simulink model "IEEE9BusSystem_eval"  (R2024a)
settings: Solver=FixedStepAuto  StartTime=0  StopTime=100  FixedStep=Ts  RelTol=1e-3  AbsTol=1e-3  EnableMultiTasking=on
PreLoadFcn:
  | Ts = 1/60;
libraries: ee_lib x63, nesl_utility x48, fl_lib x22, eeGeneralControl x6, spsFrequencyPhasorLib x3, eeSmAC1C x3, eeSmPSS1A x3, spspowerguiLib x1
(part 1 of 2)
Description:
  | IEEE 9-Bus System
settings Model: Creator=The MathWorks, Inc.  LastModifiedBy=yushixuan
settings SolverCC: AutoScaleAbsTol=off  AlgebraicLoopSolver=TrustRegion
settings DataIOCC: MaxDataPoints=110000  SaveOutput=off  DSMLogging=off  SaveTime=off  ReturnWorkspaceOutputs=off  SignalLoggingName=logsout_IEEE9BusLoadflow
settings OptimizationCC: ReuseModelBlockBuffer=off  LifeSpan=inf
settings DebuggingCC: UnderspecifiedInitializationDetection=Classic  MergeDetectMultiDrivingBlocksExec=none  MaxConsecutiveZCsMsg=warning  UnconnectedInputMsg=warning  UnconnectedOutputMsg=warning  UnconnectedLineMsg=warning  SFUnexpectedBacktrackingDiag=warning  SFNoUnconditionalDefaultTransitionDiag=warning  SFExecutionAtInitializationDiag=none  ArithmeticOperatorsInVariantConditions=warning
settings ModelReferenceCC: EnableRefExpFcnMdlSchedulingChecks=on
settings SFSimCC: SimUseLocalCustomCode=off
settings RTWCC: RTWUseLocalCustomCode=off  GPUComputeCapability=3.5
settings CodeAppCC: StateflowObjectComments=on
settings GRTTargetCC: TargetLangStandard=C89/C90 (ANSI)
settings ConfigComp: CovMetricSettings=dw  CovSaveCumulativeToWorkspaceVar=on  CovSaveSingleToWorkspaceVar=on  CovExternalEMLEnable=off
settings SimscapeCC: SimscapeNormalizeSystem=off  SimscapeLogType=all  SimscapeLogName=simlog_IEEE9BusSystem  SimscapeLogLimitData=off  SimscapeOperatingPoint=op

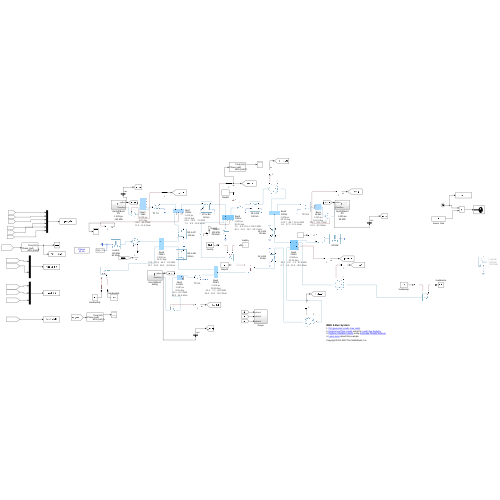
[thumbnail: Simulink's stored preview of the top-level diagram]
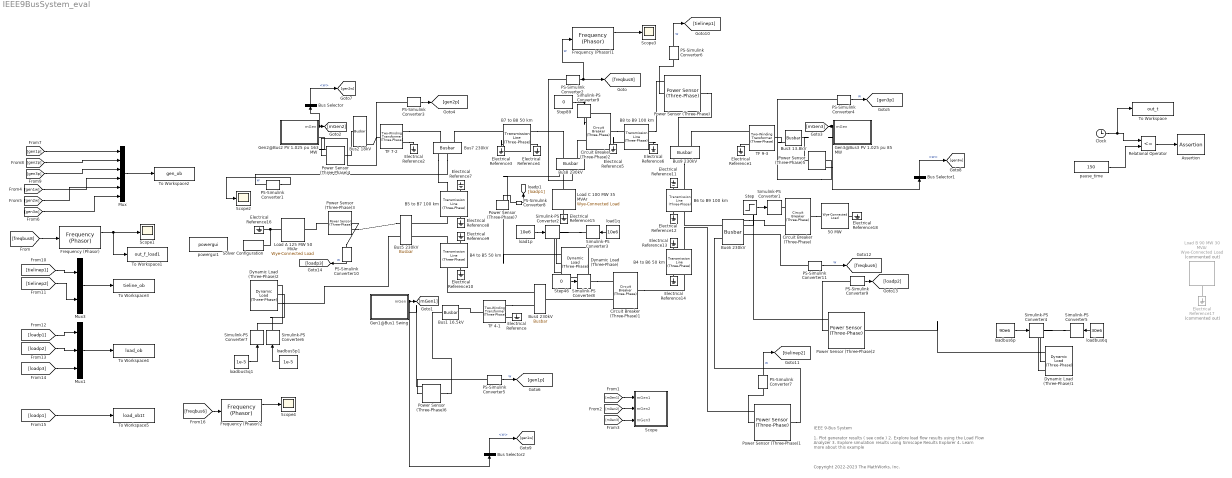
== system IEEE9BusSystem_eval ==
  note: Copyright 2022-2023 The MathWorks, Inc.
  note: 1. Plot generator results ( see code )
      | 2. Explore load flow results using the Load Flow Analyzer
      | 3. Explore simulation results using Simscape Results Explorer
      | 4. Learn more about this example
  note: IEEE 9-Bus System
  50 MW : ee_lib/Passive/RLC Assemblies/Wye-Connected Load  parameterization=2  component_structure=1  component_structure_PQ=1  R=1 Ohm  L=0.001 H  C=1e-6 F  VRated=230 kV  FRated=60 Hz  P=50 MW  Qpos=30e6 V*A  Qneg=-100 V*A  R_parasitic=1e-6 Ohm  G_parasitic=1e-6 1/Ohm  R_parasitic_PQ=1e-6 Ohm  G_parasitic_PQ=1e-6*0 1/Ohm  Vmag0=230e3 V  Vang0=0 rad  Freq0=60 Hz  IL_specify=on  IL_priority=High  IL=[ 0 0 0 ] A  IL_nominal_specify=off  IL_nominal_value=1  IL_nominal_unit=A  VC_specify=on  VC_priority=High  VC=[ 0 0 0 ] V  VC_nominal_specify=off  VC_nominal_value=1  VC_nominal_unit=V
  Assertion : Assertion  AssertionFailFcn=set_param(bdroot,'SimulationCommand','pause')  StopWhenAssertionFail=off
  B4 to B5 50 km : ee_lib/Passive/Lines/Transmission Line (Three-Phase)  length=50 km  freq=60 Hz  R=0.199333 Ohm/km  L=2.9658 mH/km  M=0.5803 mH/km  Cl=3.300e-3 uF/km  Cg=7.751e-3 uF/km  Rm=0.093533 Ohm/km  ModelTwoSections=ee.enum.enable.no  N=1  InterfacePosition=1 km  N1sec=1  N2sec=1  Access_ground=ee.enum.enable.no  R_parasitic=1e-6 Ohm  G_parasitic=1e-6 1/Ohm  EnableFault=false  fault_type_option=ee.enum.fault_type_option.ag  R_pn_fault=1e-3 Ohm  R_ng_fault=1e-3 Ohm  unfaulted_G_parasitic=1e-6 1/Ohm
      settings: InternalSimscapePortConfiguration="{\"Bottom\":[],\"Left\":[{\"id\":\"N1\",\"label\":\"~1\",\"type\":\"foundation.electrical.three_phase\"},{\"id\":\"g1\",\"label\":\"g1\",\"type\":\"foundation.electrical.electrical\"}],\"Right\":[{\"id\":\"N2\",\"label\":\"~2\",\"type\":\"foundation.electrical.three_phase\"},{\"id\":\"g2\",\"label\":\"g2\",\"type\":\"foundation.electrical.electrical\"}],\"Top\":[]}"
  B4 to B6 50 km : ee_lib/Passive/Lines/Transmission Line (Three-Phase)  length=50 km  freq=60 Hz  R=0.248707 Ohm/km  L=3.0967 mH/km  M=0.5148 mH/km  Cl=2.698e-3 uF/km  Cg=7.751e-3 uF/km  Rm=0.068847 Ohm/km  ModelTwoSections=ee.enum.enable.no  N=1  InterfacePosition=1 km  N1sec=1  N2sec=1  Access_ground=ee.enum.enable.no  R_parasitic=1e-6 Ohm  G_parasitic=1e-6 1/Ohm  EnableFault=false  fault_type_option=ee.enum.fault_type_option.ag  R_pn_fault=1e-3 Ohm  R_ng_fault=1e-3 Ohm  unfaulted_G_parasitic=1e-6 1/Ohm
      settings: InternalSimscapePortConfiguration="{\"Bottom\":[],\"Left\":[{\"id\":\"N1\",\"label\":\"~1\",\"type\":\"foundation.electrical.three_phase\"},{\"id\":\"g1\",\"label\":\"g1\",\"type\":\"foundation.electrical.electrical\"}],\"Right\":[{\"id\":\"N2\",\"label\":\"~2\",\"type\":\"foundation.electrical.three_phase\"},{\"id\":\"g2\",\"label\":\"g2\",\"type\":\"foundation.electrical.electrical\"}],\"Top\":[]}"
  B5 to B7 100 km : ee_lib/Passive/Lines/Transmission Line (Three-Phase)  length=100 km  freq=60 Hz  R=0.24165 Ohm/km  L=2.8816 mH/km  M=0.6224 mH/km  Cl=2.531e-3 uF/km  Cg=7.751e-3 uF/km  Rm=0.07237 Ohm/km  ModelTwoSections=ee.enum.enable.no  N=1  InterfacePosition=1 km  N1sec=1  N2sec=1  Access_ground=ee.enum.enable.no  R_parasitic=1e-6 Ohm  G_parasitic=1e-6 1/Ohm  EnableFault=false  fault_type_option=ee.enum.fault_type_option.ag  R_pn_fault=1e-3 Ohm  R_ng_fault=1e-3 Ohm  unfaulted_G_parasitic=1e-6 1/Ohm
      settings: InternalSimscapePortConfiguration="{\"Bottom\":[],\"Left\":[{\"id\":\"N1\",\"label\":\"~1\",\"type\":\"foundation.electrical.three_phase\"},{\"id\":\"g1\",\"label\":\"g1\",\"type\":\"foundation.electrical.electrical\"}],\"Right\":[{\"id\":\"N2\",\"label\":\"~2\",\"type\":\"foundation.electrical.three_phase\"},{\"id\":\"g2\",\"label\":\"g2\",\"type\":\"foundation.electrical.electrical\"}],\"Top\":[]}"
  B6 to B9 100 km : ee_lib/Passive/Lines/Transmission Line (Three-Phase)  length=100 km  freq=60 Hz  R=0.26634 Ohm/km  L=2.9658 mH/km  M=0.5803 mH/km  Cl=3.400e-3 uF/km  Cg=7.751e-3 uF/km  Rm=0.06003 Ohm/km  ModelTwoSections=ee.enum.enable.no  N=1  InterfacePosition=1 km  N1sec=1  N2sec=1  Access_ground=ee.enum.enable.no  R_parasitic=1e-6 Ohm  G_parasitic=1e-6 1/Ohm  EnableFault=false  fault_type_option=ee.enum.fault_type_option.ag  R_pn_fault=1e-3 Ohm  R_ng_fault=1e-3 Ohm  unfaulted_G_parasitic=1e-6 1/Ohm
      settings: InternalSimscapePortConfiguration="{\"Bottom\":[],\"Left\":[{\"id\":\"N1\",\"label\":\"~1\",\"type\":\"foundation.electrical.three_phase\"},{\"id\":\"g1\",\"label\":\"g1\",\"type\":\"foundation.electrical.electrical\"}],\"Right\":[{\"id\":\"N2\",\"label\":\"~2\",\"type\":\"foundation.electrical.three_phase\"},{\"id\":\"g2\",\"label\":\"g2\",\"type\":\"foundation.electrical.electrical\"}],\"Top\":[]}"
  B7 to B8 50 km : ee_lib/Passive/Lines/Transmission Line (Three-Phase)  length=50 km  freq=60 Hz  R=0.18875 Ohm/km  L=2.7226 mH/km  M=0.7019 mH/km  Cl=2.731e-3 uF/km  Cg=6.751e-3 uF/km  Rm=0.09882 Ohm/km  ModelTwoSections=ee.enum.enable.no  N=1  InterfacePosition=1 km  N1sec=1  N2sec=1  Access_ground=ee.enum.enable.no  R_parasitic=1e-6 Ohm  G_parasitic=1e-6 1/Ohm  EnableFault=false  fault_type_option=ee.enum.fault_type_option.ag  R_pn_fault=1e-3 Ohm  R_ng_fault=1e-3 Ohm  unfaulted_G_parasitic=1e-6 1/Ohm
      settings: InternalSimscapePortConfiguration="{\"Bottom\":[],\"Left\":[{\"id\":\"N1\",\"label\":\"~1\",\"type\":\"foundation.electrical.three_phase\"},{\"id\":\"g1\",\"label\":\"g1\",\"type\":\"foundation.electrical.electrical\"}],\"Right\":[{\"id\":\"N2\",\"label\":\"~2\",\"type\":\"foundation.electrical.three_phase\"},{\"id\":\"g2\",\"label\":\"g2\",\"type\":\"foundation.electrical.electrical\"}],\"Top\":[]}"
  B8 to B9 100 km : ee_lib/Passive/Lines/Transmission Line (Three-Phase)  length=100 km  freq=60 Hz  R=0.17077 Ohm/km  L=2.3184 mH/km  M=0.9040 mH/km  Cl=9.097e-4 uF/km  Cg=7.751e-3 uF/km  Rm=0.10782 Ohm/km  ModelTwoSections=ee.enum.enable.no  N=1  InterfacePosition=1 km  N1sec=1  N2sec=1  Access_ground=ee.enum.enable.no  R_parasitic=1e-6 Ohm  G_parasitic=1e-6 1/Ohm  EnableFault=false  fault_type_option=ee.enum.fault_type_option.ag  R_pn_fault=1e-3 Ohm  R_ng_fault=1e-3 Ohm  unfaulted_G_parasitic=1e-6 1/Ohm
      settings: InternalSimscapePortConfiguration="{\"Bottom\":[],\"Left\":[{\"id\":\"N1\",\"label\":\"~1\",\"type\":\"foundation.electrical.three_phase\"},{\"id\":\"g1\",\"label\":\"g1\",\"type\":\"foundation.electrical.electrical\"}],\"Right\":[{\"id\":\"N2\",\"label\":\"~2\",\"type\":\"foundation.electrical.three_phase\"},{\"id\":\"g2\",\"label\":\"g2\",\"type\":\"foundation.electrical.electrical\"}],\"Top\":[]}"
  Bus Selector : BusSelector  OutputSignals=w
  Bus Selector1 : BusSelector  OutputSignals=w
  Bus Selector2 : BusSelector  OutputSignals=w
  Bus1 16.5kV : ee_lib/Connectors & References/Busbar  Tag="1.040 pu\\n0.00 deg\\n42.4  -42.4 MW\\n38.5  -38.5 Mvar"  n_nodes=ee.enum.connectors.busbar_number_of_connections.two  VRated=16.5 kV  freq=60 Hz  show_ps=ee.enum.connectors.busbar_measurement.true
      settings: AttributesFormatString=%<Tag>  InternalSimscapePortConfiguration="{\"Bottom\":[],\"Left\":[{\"id\":\"N1\",\"label\":\"~1\",\"type\":\"foundation.electrical.three_phase\"}],\"Right\":[{\"id\":\"N2\",\"label\":\"~2\",\"type\":\"foundation.electrical.three_phase\"},{\"id\":\"Vt_ps\",\"label\":\"Vt\",\"type\":\"output\"},{\"id\":\"ph_ps\",\"label\":\"ph\",\"type\":\"output\"},{\"id\":\"P2_ps\",\"label\":\"P\",\"type\":\"output\"},{\"id\":\"Q2_ps\",\"label\":\"Q\",\"type\":\"output\"}],\"Top\":[]}"
  Bus2 18kV : ee_lib/Connectors & References/Busbar  Tag="1.025 pu\\n6.07 deg\\n83.2  -83.2 MW\\n11.5  -11.5 Mvar"  n_nodes=ee.enum.connectors.busbar_number_of_connections.two  VRated=18 kV  freq=60 Hz  show_ps=ee.enum.connectors.busbar_measurement.true
      settings: AttributesFormatString=%<Tag>  InternalSimscapePortConfiguration="{\"Bottom\":[],\"Left\":[{\"id\":\"N1\",\"label\":\"~1\",\"type\":\"foundation.electrical.three_phase\"}],\"Right\":[{\"id\":\"N2\",\"label\":\"~2\",\"type\":\"foundation.electrical.three_phase\"},{\"id\":\"Vt_ps\",\"label\":\"Vt\",\"type\":\"output\"},{\"id\":\"ph_ps\",\"label\":\"ph\",\"type\":\"output\"},{\"id\":\"P2_ps\",\"label\":\"P\",\"type\":\"output\"},{\"id\":\"Q2_ps\",\"label\":\"Q\",\"type\":\"output\"}],\"Top\":[]}"
  Bus3 13.8kV : ee_lib/Connectors & References/Busbar  Tag="1.025 pu\\n15.16 deg\\n201.7 -201.7 MW\\n10.9  -10.9 Mvar"  n_nodes=ee.enum.connectors.busbar_number_of_connections.two  VRated=13.8 kV  freq=60 Hz  show_ps=ee.enum.connectors.busbar_measurement.true
      settings: AttributesFormatString=%<Tag>  InternalSimscapePortConfiguration="{\"Bottom\":[],\"Left\":[{\"id\":\"N1\",\"label\":\"~1\",\"type\":\"foundation.electrical.three_phase\"}],\"Right\":[{\"id\":\"N2\",\"label\":\"~2\",\"type\":\"foundation.electrical.three_phase\"},{\"id\":\"Vt_ps\",\"label\":\"Vt\",\"type\":\"output\"},{\"id\":\"ph_ps\",\"label\":\"ph\",\"type\":\"output\"},{\"id\":\"P2_ps\",\"label\":\"P\",\"type\":\"output\"},{\"id\":\"Q2_ps\",\"label\":\"Q\",\"type\":\"output\"}],\"Top\":[]}"
  Bus4 230kV : ee_lib/Connectors & References/Busbar  Tag="1.019 pu\\n28.69 deg\\n42.2    7.2  -49.4 MW\\n36.5  -16.3  -20.2 Mvar"  n_nodes=ee.enum.connectors.busbar_number_of_connections.three  VRated=230 kV  freq=60 Hz  show_ps=ee.enum.connectors.busbar_measurement.false
      settings: AttributesFormatString=%<Tag>  InternalSimscapePortConfiguration="{\"Bottom\":[],\"Left\":[{\"id\":\"N1\",\"label\":\"~1\",\"type\":\"foundation.electrical.three_phase\"},{\"id\":\"N3\",\"label\":\"~3\",\"type\":\"foundation.electrical.three_phase\"}],\"Right\":[{\"id\":\"N2\",\"label\":\"~2\",\"type\":\"foundation.electrical.three_phase\"}],\"Top\":[]}"
  Bus5 230kV : ee_lib/Connectors & References/Busbar  Tag="0.990 pu\\n26.47 deg\\n73.5 -122.6   49.1   -0.0 MW\\n13.7  -49.0   35.3   -0.0 Mvar"  n_nodes=ee.enum.connectors.busbar_number_of_connections.four  VRated=230 kV  freq=60 Hz  show_ps=ee.enum.connectors.busbar_measurement.false
      settings: AttributesFormatString=%<Tag>  InternalSimscapePortConfiguration="{\"Bottom\":[],\"Left\":[{\"id\":\"N1\",\"label\":\"~1\",\"type\":\"foundation.electrical.three_phase\"},{\"id\":\"N3\",\"label\":\"~3\",\"type\":\"foundation.electrical.three_phase\"}],\"Right\":[{\"id\":\"N2\",\"label\":\"~2\",\"type\":\"foundation.electrical.three_phase\"},{\"id\":\"N4\",\"label\":\"~4\",\"type\":\"foundation.electrical.three_phase\"}],\"Top\":[]}"
  Bus6 230kV : ee_lib/Connectors & References/Busbar  Tag="0.998 pu\\n29.30 deg\\n95.1   -0.0   -7.3  -87.8 MW\\n3.7   -0.0   31.8  -35.5 Mvar"  n_nodes=ee.enum.connectors.busbar_number_of_connections.four  VRated=230 kV  freq=60 Hz  show_ps=ee.enum.connectors.busbar_measurement.true
      settings: AttributesFormatString=%<Tag>  InternalSimscapePortConfiguration="{\"Bottom\":[],\"Left\":[{\"id\":\"N1\",\"label\":\"~1\",\"type\":\"foundation.electrical.three_phase\"},{\"id\":\"N3\",\"label\":\"~3\",\"type\":\"foundation.electrical.three_phase\"}],\"Right\":[{\"id\":\"N2\",\"label\":\"~2\",\"type\":\"foundation.electrical.three_phase\"},{\"id\":\"N4\",\"label\":\"~4\",\"type\":\"foundation.electrical.three_phase\"},{\"id\":\"Vt_ps\",\"label\":\"Vt\",\"type\":\"output\"},{\"id\":\"ph_ps\",\"label\":\"ph\",\"type\":\"output\"},{\"id\":\"P4_ps\",\"label\":\"P\",\"type\":\"output\"},{\"id\":\"Q4_ps\",\"label\":\"Q\",\"type\":\"output\"}],\"Top\":[]}"
  Bus7 230kV : ee_lib/Connectors & References/Busbar  Tag="1.019 pu\\n33.23 deg\\n82.9  -75.3   -7.6 MW\\n7.2    8.3  -15.4 Mvar"  n_nodes=ee.enum.connectors.busbar_number_of_connections.three  VRated=230 kV  freq=60 Hz  show_ps=ee.enum.connectors.busbar_measurement.true
      settings: AttributesFormatString=%<Tag>  InternalSimscapePortConfiguration="{\"Bottom\":[],\"Left\":[{\"id\":\"N1\",\"label\":\"~1\",\"type\":\"foundation.electrical.three_phase\"},{\"id\":\"N3\",\"label\":\"~3\",\"type\":\"foundation.electrical.three_phase\"}],\"Right\":[{\"id\":\"N2\",\"label\":\"~2\",\"type\":\"foundation.electrical.three_phase\"},{\"id\":\"Vt_ps\",\"label\":\"Vt\",\"type\":\"output\"},{\"id\":\"ph_ps\",\"label\":\"ph\",\"type\":\"output\"},{\"id\":\"P3_ps\",\"label\":\"P\",\"type\":\"output\"},{\"id\":\"Q3_ps\",\"label\":\"Q\",\"type\":\"output\"}],\"Top\":[]}"
  Bus8 230kV : ee_lib/Connectors & References/Busbar  Tag="1.002 pu\\n33.03 deg\\n7.6   -8.6  101.4 -100.5 MW\\n30.2  -11.3   16.2  -35.1 Mvar"  n_nodes=ee.enum.connectors.busbar_number_of_connections.four  VRated=230 kV  freq=60 Hz  show_ps=ee.enum.connectors.busbar_measurement.true
      settings: AttributesFormatString=%<Tag>  InternalSimscapePortConfiguration="{\"Bottom\":[],\"Left\":[{\"id\":\"N1\",\"label\":\"~1\",\"type\":\"foundation.electrical.three_phase\"},{\"id\":\"N3\",\"label\":\"~3\",\"type\":\"foundation.electrical.three_phase\"}],\"Right\":[{\"id\":\"N2\",\"label\":\"~2\",\"type\":\"foundation.electrical.three_phase\"},{\"id\":\"N4\",\"label\":\"~4\",\"type\":\"foundation.electrical.three_phase\"},{\"id\":\"Vt_ps\",\"label\":\"Vt\",\"type\":\"output\"},{\"id\":\"ph_ps\",\"label\":\"ph\",\"type\":\"output\"},{\"id\":\"P4_ps\",\"label\":\"P\",\"type\":\"output\"},{\"id\":\"Q4_ps\",\"label\":\"Q\",\"type\":\"output\"}],\"Top\":[]}"
  Bus9 230kV : ee_lib/Connectors & References/Busbar  Tag="1.025 pu\\n38.70 deg\\n-102.7  -98.7  201.4 MW\\n-5.1   17.2  -12.1 Mvar"  n_nodes=ee.enum.connectors.busbar_number_of_connections.three  VRated=230 kV  freq=60 Hz  show_ps=ee.enum.connectors.busbar_measurement.false
      settings: AttributesFormatString=%<Tag>  InternalSimscapePortConfiguration="{\"Bottom\":[],\"Left\":[{\"id\":\"N1\",\"label\":\"~1\",\"type\":\"foundation.electrical.three_phase\"},{\"id\":\"N3\",\"label\":\"~3\",\"type\":\"foundation.electrical.three_phase\"}],\"Right\":[{\"id\":\"N2\",\"label\":\"~2\",\"type\":\"foundation.electrical.three_phase\"}],\"Top\":[]}"
  Circuit Breaker (Three-Phase) : ee_lib/Switches & Breakers/Circuit Breaker (Three-Phase)  R_closed=0.001 Ohm  G_open=1e-8 1/Ohm  threshold=0.5 V  breaker_behavior=ee.enum.switches.breakerBehavior.zeroCrossingDisable
      settings: InternalSimscapePortConfiguration="{\"Bottom\":[],\"Left\":[{\"id\":\"vT\",\"label\":\"vT\",\"type\":\"input\"},{\"id\":\"N1\",\"label\":\"~1\",\"type\":\"foundation.electrical.three_phase\"}],\"Right\":[{\"id\":\"N2\",\"label\":\"~2\",\"type\":\"foundation.electrical.three_phase\"}],\"Top\":[]}"
  Circuit Breaker (Three-Phase)1 : ee_lib/Switches & Breakers/Circuit Breaker (Three-Phase)  R_closed=0.001 Ohm  G_open=1e-8 1/Ohm  threshold=0.5 V  breaker_behavior=ee.enum.switches.breakerBehavior.zeroCrossingDisable
      settings: InternalSimscapePortConfiguration="{\"Bottom\":[],\"Left\":[{\"id\":\"vT\",\"label\":\"vT\",\"type\":\"input\"},{\"id\":\"N1\",\"label\":\"~1\",\"type\":\"foundation.electrical.three_phase\"}],\"Right\":[{\"id\":\"N2\",\"label\":\"~2\",\"type\":\"foundation.electrical.three_phase\"}],\"Top\":[]}"
  Circuit Breaker (Three-Phase)2 : ee_lib/Switches & Breakers/Circuit Breaker (Three-Phase)  R_closed=0.001 Ohm  G_open=1e-8 1/Ohm  threshold=0.5 V  breaker_behavior=ee.enum.switches.breakerBehavior.zeroCrossingDisable
      settings: InternalSimscapePortConfiguration="{\"Bottom\":[],\"Left\":[{\"id\":\"vT\",\"label\":\"vT\",\"type\":\"input\"},{\"id\":\"N1\",\"label\":\"~1\",\"type\":\"foundation.electrical.three_phase\"}],\"Right\":[{\"id\":\"N2\",\"label\":\"~2\",\"type\":\"foundation.electrical.three_phase\"}],\"Top\":[]}"
  Clock : Clock
  Dynamic Load (Three-Phase) : ee_lib/Passive/Dynamic Load (Three-Phase)  port_option=ee.enum.threePhasePort.composite  FRated=60 Hz  Vline_rms_min=230e3 V  tau=0.01 s  Vline_rms_ini=230e3 V  Vang_ini=25.2 deg  gmin=0 S  enable_fault=simscape.enum.onoff.off  fault_action=simscape.enum.assert.action.none  t_fault=1 s  open_conductance=1e-4 S
      settings: InternalSimscapePortConfiguration="{\"Bottom\":[],\"Left\":[{\"id\":\"N\",\"label\":\"~\",\"type\":\"foundation.electrical.three_phase\"}],\"Right\":[],\"Top\":[{\"id\":\"P\",\"label\":\"P\",\"type\":\"input\"},{\"id\":\"Q\",\"label\":\"Q\",\"type\":\"input\"}]}"
  Dynamic Load (Three-Phase)1 : ee_lib/Passive/Dynamic Load (Three-Phase)  port_option=ee.enum.threePhasePort.composite  FRated=60 Hz  Vline_rms_min=230e3 V  tau=0.01 s  Vline_rms_ini=230e3 V  Vang_ini=25.71 deg  gmin=0 S  enable_fault=simscape.enum.onoff.off  fault_action=simscape.enum.assert.action.none  t_fault=1 s  open_conductance=1e-4 S
      settings: InternalSimscapePortConfiguration="{\"Bottom\":[],\"Left\":[{\"id\":\"N\",\"label\":\"~\",\"type\":\"foundation.electrical.three_phase\"}],\"Right\":[],\"Top\":[{\"id\":\"P\",\"label\":\"P\",\"type\":\"input\"},{\"id\":\"Q\",\"label\":\"Q\",\"type\":\"input\"}]}"
  Dynamic Load (Three-Phase)2 : ee_lib/Passive/Dynamic Load (Three-Phase)  port_option=ee.enum.threePhasePort.composite  FRated=60 Hz  Vline_rms_min=230e3 V  tau=0.01 s  Vline_rms_ini=230e3 V  Vang_ini=25.46 deg  gmin=0 S  enable_fault=simscape.enum.onoff.off  fault_action=simscape.enum.assert.action.none  t_fault=1 s  open_conductance=1e-4 S
      settings: InternalSimscapePortConfiguration="{\"Bottom\":[],\"Left\":[{\"id\":\"N\",\"label\":\"~\",\"type\":\"foundation.electrical.three_phase\"}],\"Right\":[],\"Top\":[{\"id\":\"P\",\"label\":\"P\",\"type\":\"input\"},{\"id\":\"Q\",\"label\":\"Q\",\"type\":\"input\"}]}"
  Electrical Reference{,1..16,18} (18 alike) : fl_lib/Electrical/Electrical Elements/Electrical Reference
  Electrical Reference17 : fl_lib/Electrical/Electrical Elements/Electrical Reference  Commented=on
  Frequency (Phasor) : spsFrequencyPhasorLib/Frequency (Phasor)  Fn=60  T=0.1
      settings: LibrarySourceBlock=|
      | sps_lib/Sensors and Measurements/Frequency
      | (Phasor)
  Frequency (Phasor)1 : spsFrequencyPhasorLib/Frequency (Phasor)  Fn=60  T=0.1
      settings: LibrarySourceBlock=|
      | sps_lib/Sensors and Measurements/Frequency
      | (Phasor)
  Frequency (Phasor)2 : spsFrequencyPhasorLib/Frequency (Phasor)  Fn=60  T=0.1
      settings: LibrarySourceBlock=|
      | sps_lib/Sensors and Measurements/Frequency
      | (Phasor)
  Gen1@Bus1 Swing : Subsystem
  Gen2@Bus2 PV 1.025 pu 163 MW : Subsystem
  Gen3@Bus3 PV 1.025 pu 85 MW : Subsystem
  Load A 125 MW 50 MVAr : ee_lib/Passive/RLC Assemblies/Wye-Connected Load  parameterization=2  component_structure=1  component_structure_PQ=4  R=1 Ohm  L=0.001 H  C=1e-6 F  VRated=230e3 V  FRated=60 Hz  P=125e6 W  Qpos=50e6 V*A  Qneg=-100 V*A  R_parasitic=1e-6 Ohm  G_parasitic=1e-6 1/Ohm  R_parasitic_PQ=1e-6 Ohm  G_parasitic_PQ=1e-6 1/Ohm  Vmag0=230e3 V  Vang0=0 deg  Freq0=60 Hz  IL_specify=on  IL_priority=High  IL=[ 0 0 0 ] A  IL_nominal_specify=off  IL_nominal_value=1  IL_nominal_unit=A  VC_specify=on  VC_priority=High  VC=[ 0 0 0 ] V  VC_nominal_specify=off  VC_nominal_value=1  VC_nominal_unit=V
  Load B 90 MW 30 MVAr : ee_lib/Passive/RLC Assemblies/Wye-Connected Load  Commented=on  parameterization=2  component_structure=1  component_structure_PQ=4  R=1 Ohm  L=0.001 H  C=1e-6 F  VRated=230e3 V  FRated=60 Hz  P=90e6 W  Qpos=30e6 V*A  Qneg=-100 V*A  R_parasitic=1e-6 Ohm  G_parasitic=1e-6 1/Ohm  R_parasitic_PQ=1e-6 Ohm  G_parasitic_PQ=1e-6*0 1/Ohm  Vmag0=230e3 V  Vang0=0 deg  Freq0=60 Hz  IL_specify=on  IL_priority=High  IL=[ 0 0 0 ] A  IL_nominal_specify=off  IL_nominal_value=1  IL_nominal_unit=A  VC_specify=on  VC_priority=High  VC=[ 0 0 0 ] V  VC_nominal_specify=off  VC_nominal_value=1  VC_nominal_unit=V
  Load C 100 MW 35 MVAr : ee_lib/Passive/RLC Assemblies/Wye-Connected Load  parameterization=2  component_structure=1  component_structure_PQ=4  R=1 Ohm  L=0.001 H  C=1e-6 F  VRated=230e3 V  FRated=60 Hz  P=100e6 W  Qpos=35e6 V*A  Qneg=-100 V*A  R_parasitic=1e-6 Ohm  G_parasitic=1e-6 1/Ohm  R_parasitic_PQ=1e-6 Ohm  G_parasitic_PQ=1e-6 1/Ohm  Vmag0=230e3 V  Vang0=0 deg  Freq0=60 Hz  IL_specify=on  IL_priority=High  IL=[ 0 0 0 ] A  IL_nominal_specify=off  IL_nominal_value=1  IL_nominal_unit=A  VC_specify=on  VC_priority=High  VC=[ 0 0 0 ] V  VC_nominal_specify=off  VC_nominal_value=1  VC_nominal_unit=V
  Mux : Mux  Inputs=6
  Mux1 : Mux  Inputs=3
  Mux3 : Mux  Inputs=2
  PS-Simulink Converter{1..11} (11 alike) : nesl_utility/PS-Simulink Converter  PhysicalDomain=network_engine_domain  SubClassName=ps_output  LeftPortType=input  RightPortType=output  PseudoPeriodic=off  Frequencies=[]  VectorFormat=1-D array  Unit=1  AffineConversion=off
  Power Sensor (Three-Phase){,1..7} (8 alike) : ee_lib/Sensors & Transducers/Power Sensor (Three-Phase)  load_type=ee.enum.passive.type_balanced.balanced  f0=60 Hz  config=ee.enum.with_neutral.no  rho=1
      settings: InternalSimscapePortConfiguration="{\"Bottom\":[],\"Left\":[{\"id\":\"N1\",\"label\":\"~1\",\"type\":\"foundation.electrical.three_phase\"}],\"Right\":[{\"id\":\"N2\",\"label\":\"~2\",\"type\":\"foundation.electrical.three_phase\"}],\"Top\":[{\"id\":\"Pm\",\"label\":\"P\",\"type\":\"output\"},{\"id\":\"Qm\",\"label\":\"Q\",\"type\":\"output\"}]}"
  Relational Operator : RelationalOperator  Operator=<=  OutDataTypeStr=boolean  RndMeth=Simplest  InputSameDT=off
  Scope : Subsystem
  Scope{1..4} (4 alike) : Scope
  Simulink-PS Converter{1..9} (9 alike) : nesl_utility/Simulink-PS Converter  PhysicalDomain=network_engine_domain  SubClassName=ps_input  LeftPortType=input  RightPortType=output  PseudoPeriodic=off  Frequencies=[]  NoiseDistribution=none  NoiseParameters=[]  Unit=1  AffineConversion=off  FilteringAndDerivatives=provide  SimscapeFilterOrder=1  InputFilterTimeConstant=0.001  UdotUserProvided=0
  Solver Configuration : nesl_utility/Solver Configuration  PhysicalDomain=network_engine_domain  SubClassName=solver  LeftPortType=input  RightPortType=generic  Tones=[]  Harmonics=[]  SimulateNoise=off  Profile=off  UseLocalSampling=off  EnableSwitchedLinearOptims=on  FrequencyDomain=off  UseCCode=off  RelTol=0.001  AbsTol=1e-06  MinStep=1e-09  ToWorkspace=off  RevertToSquareIcSolve=off  NumHomotopyIterations=100  PhasorMode=off  PhasorModeNumHarmonics=1  ConsistencySolver=NEWTON_FTOL  IndexReductionMethod=DerivativeReplacement  DoDC=off  ResidualTolerance=1e-09  ConsistencyTolSource=GLOBAL  ConsistencyAbsTol=0.001  ConsistencyRelTol=0.001  ConsistencyTolFactor=0.001  UseLocalSolver=on  LocalSolverChoice=NE_BACKWARD_EULER_ADVANCER  ResolveIndetEquations=on  FunctionEvalNumThread=1  LocalSolverSampleTime=Ts  DoFixedCost=on  MaxNonlinIter=3  MaxModeIter=2  ComputeImpulses=off  ImpulseIterations=2  LinearAlgebra=auto  LinearAlgebraNumThread=0  EquationFormulation=NE_FREQUENCY_TIME_EF  DelaysMemoryBudget=1024  AutomaticFiltering=on  FilteringTimeConstant=0.001  PartitionStorageMethod=AS_NEEDED  PartitionMemoryBudget=1024  PartitionMethod=FAST  MultibodyUseLocalSolver=off  MultibodyLocalSolverChoice=ODE1  MultibodyLocalSolverSampleTime=0.001
  Step : Step  Time=150  Before=1  After=0  SampleTime=0
  Step46 : Constant  Value=0
  Step89 : Constant  Value=0
  TF 4-1 : ee_lib/Passive/Transformers/Two-Winding Transformer (Three-Phase)  SRated=100e6 V*A  FRated=60 Hz  Winding1Connection=ee.enum.windingconnection.Yn  VRated1=230e3 V  Winding2Connection=ee.enum.windingconnection.delta1  VRated2=16.5e3 V  CoreType=ee.enum.coretype.fivelimb  pu_Rw1=1e-4  pu_Rw2=1e-4  leakage_reactance_option=ee.enum.transformer_leakage.include  pu_Xl1=0.0576/2  pu_Xl2=0.0576/2  magnetizing_resistance_option=ee.enum.transformer_magnetizingResistance.include  pu_Rm=500  magnetizing_reactance_option=ee.enum.transformer_magnetizingReactance.include  saturation_option=ee.enum.transformer_saturation.exclude  pu_Xm=500  current_data=[0, .002, 1, 2]  magnetic_flux_data=[0, 1.2, 1.5, 1.51]  pu_X0=0.5  i1_specify=off  i1_priority=None  i1=[ 0 0 0 ] A  i1_nominal_specify=off  i1_nominal_value=1  i1_nominal_unit=A  i2_specify=off  i2_priority=None  i2=[ 0 0 0 ] A  i2_nominal_specify=off  i2_nominal_value=1  i2_nominal_unit=A  phi_specify=off  phi_priority=None  phi=[ 0 0 0 ]  phi_nominal_specify=off  phi_nominal_value=1  phi_nominal_unit=1  power_dissipated_specify=off  power_dissipated_priority=None  power_dissipated=0 W  power_dissipated_nominal_specify=off  power_dissipated_nominal_value=1  power_dissipated_nominal_unit=W
      settings: InternalSimscapePortConfiguration="{\"Bottom\":[],\"Left\":[{\"id\":\"N1\",\"label\":\"~1\",\"type\":\"foundation.electrical.three_phase\"},{\"id\":\"n1\",\"label\":\"n1\",\"type\":\"foundation.electrical.electrical\"}],\"Right\":[{\"id\":\"N2\",\"label\":\"~2\",\"type\":\"foundation.electrical.three_phase\"}],\"Top\":[]}"
  TF 7-2 : ee_lib/Passive/Transformers/Two-Winding Transformer (Three-Phase)  SRated=100e6 V*A  FRated=60 Hz  Winding1Connection=ee.enum.windingconnection.Yn  VRated1=230e3 V  Winding2Connection=ee.enum.windingconnection.delta1  VRated2=18e3 V  CoreType=ee.enum.coretype.fivelimb  pu_Rw1=1e-4  pu_Rw2=1e-4  leakage_reactance_option=ee.enum.transformer_leakage.include  pu_Xl1=0.0625/2  pu_Xl2=0.0625/2  magnetizing_resistance_option=ee.enum.transformer_magnetizingResistance.include  pu_Rm=500  magnetizing_reactance_option=ee.enum.transformer_magnetizingReactance.include  saturation_option=ee.enum.transformer_saturation.exclude  pu_Xm=500  current_data=[0, .002, 1, 2]  magnetic_flux_data=[0, 1.2, 1.5, 1.51]  pu_X0=0.5  i1_specify=off  i1_priority=None  i1=[ 0 0 0 ] A  i1_nominal_specify=off  i1_nominal_value=1  i1_nominal_unit=A  i2_specify=off  i2_priority=None  i2=[ 0 0 0 ] A  i2_nominal_specify=off  i2_nominal_value=1  i2_nominal_unit=A  phi_specify=off  phi_priority=None  phi=[ 0 0 0 ]  phi_nominal_specify=off  phi_nominal_value=1  phi_nominal_unit=1  power_dissipated_specify=off  power_dissipated_priority=None  power_dissipated=0 W  power_dissipated_nominal_specify=off  power_dissipated_nominal_value=1  power_dissipated_nominal_unit=W
      settings: InternalSimscapePortConfiguration="{\"Bottom\":[],\"Left\":[{\"id\":\"N1\",\"label\":\"~1\",\"type\":\"foundation.electrical.three_phase\"},{\"id\":\"n1\",\"label\":\"n1\",\"type\":\"foundation.electrical.electrical\"}],\"Right\":[{\"id\":\"N2\",\"label\":\"~2\",\"type\":\"foundation.electrical.three_phase\"}],\"Top\":[]}"
  TF 9-3 : ee_lib/Passive/Transformers/Two-Winding Transformer (Three-Phase)  SRated=100e6 V*A  FRated=60 Hz  Winding1Connection=ee.enum.windingconnection.Yn  VRated1=230e3 V  Winding2Connection=ee.enum.windingconnection.delta1  VRated2=13.8e3 V  CoreType=ee.enum.coretype.fivelimb  pu_Rw1=1e-4  pu_Rw2=1e-4  leakage_reactance_option=ee.enum.transformer_leakage.include  pu_Xl1=0.0586/2  pu_Xl2=0.0586/2  magnetizing_resistance_option=ee.enum.transformer_magnetizingResistance.include  pu_Rm=500  magnetizing_reactance_option=ee.enum.transformer_magnetizingReactance.include  saturation_option=ee.enum.transformer_saturation.exclude  pu_Xm=500  current_data=[0, .002, 1, 2]  magnetic_flux_data=[0, 1.2, 1.5, 1.51]  pu_X0=0.5  i1_specify=off  i1_priority=None  i1=[ 0 0 0 ] A  i1_nominal_specify=off  i1_nominal_value=1  i1_nominal_unit=A  i2_specify=off  i2_priority=None  i2=[ 0 0 0 ] A  i2_nominal_specify=off  i2_nominal_value=1  i2_nominal_unit=A  phi_specify=off  phi_priority=None  phi=[ 0 0 0 ]  phi_nominal_specify=off  phi_nominal_value=1  phi_nominal_unit=1  power_dissipated_specify=off  power_dissipated_priority=None  power_dissipated=0 W  power_dissipated_nominal_specify=off  power_dissipated_nominal_value=1  power_dissipated_nominal_unit=W
      settings: InternalSimscapePortConfiguration="{\"Bottom\":[],\"Left\":[{\"id\":\"N1\",\"label\":\"~1\",\"type\":\"foundation.electrical.three_phase\"},{\"id\":\"n1\",\"label\":\"n1\",\"type\":\"foundation.electrical.electrical\"}],\"Right\":[{\"id\":\"N2\",\"label\":\"~2\",\"type\":\"foundation.electrical.three_phase\"}],\"Top\":[]}"
  To Workspace : ToWorkspace  VariableName=out_t  SampleTime=0.2
      settings: Save2DSignal=2-D array (concatenate along first dimension)
  To Workspace1 : ToWorkspace  VariableName=out_f_load1  SampleTime=0.2
  To Workspace2 : ToWorkspace  VariableName=gen_ob  SampleTime=1
  To Workspace3 : ToWorkspace  VariableName=tieline_ob  SampleTime=1
  To Workspace4 : ToWorkspace  VariableName=load_ob  SampleTime=1
  To Workspace5 : ToWorkspace  VariableName=load_ob1t  SampleTime=0.2
  load1p : Constant  Value=10e6
  load1q : Constant  Value=10e6
  loadbus5p1 : Constant  Value=1e-5
  loadbus5q1 : Constant  Value=1e-5
  loadbus6p : Constant  Value=90e6
  loadbus6q : Constant  Value=30e6
  pause_time : Constant  Value=150
  powergui1 : spspowerguiLib/powergui  Priority=2  SimulationMode=Phasor  SampleTime=Ts  frequency=60  Iterations=50  frequencyindice=60  Pbase=100e6  ErrMax=0.0001  UnitsV=kV  UnitsW=MW  buscounter=0  FunctionMessages=off  echomessages=off  EnableUseOfTLC=off  CurrentSourceSwitches=off  DisableSnubberDevices=off  DisableRonSwitches=off  DisableVfSwitches=off  DisplayEquations=off  AutomaticDiscreteSolvers=off  SolverType=Tustin  Interpol=off  ExternalGateDelay=off  methode=off  Ts=0  x0status=blocks  SPID=off  SwTol=0  HookPort=off  NonlinearTolerance=1e-4  nMaxIteration=100  ContinueOnMaxIteration=off  RestoreLinks=warning  ResistiveCurrentMeasurement=off  Frange=logspace(0,3,50)  Ylog=off  Xlog=off  ShowGrid=off  save=off  variable=ZData  structure=0  ZoomFFT=on  StartTime=0.0  cycles=1  DisplayStyle=1  fundamental=60  FreqAxis=off  MaxFrequency=1000  frequencyindicesteady=1  RmsSteady=1  display=off
  wires:
  Gen2@Bus2 PV 1.025 pu 163 MW/1(mGen) -> Bus Selector/1, [mGen2]
  Step/1 -> Simulink-PS Converter1/1
  [mGen1] -> Scope/1(mGen1)
  [mGen2] -> Scope/2(mGen2)
  [mGen3] -> Scope/3(mGen3)
  load1p/1 -> Simulink-PS Converter2/1
  load1q/1 -> Simulink-PS Converter3/1
  pause_time/1 -> Relational Operator/2
  Relational Operator/1 -> Assertion/1
  Clock/1 -> To Workspace/1, Relational Operator/1
  PS-Simulink Converter1/1 -> Scope2/1  "w"
  PS-Simulink Converter2/1 -> Frequency (Phasor)1/1, [freqbus8]  "w"
  [freqbus8] -> Frequency (Phasor)/1
  Frequency (Phasor)/1 -> To Workspace1/1, Scope1/1
  PS-Simulink Converter4/1 -> [gen3p]  "w"
  PS-Simulink Converter5/1 -> [gen1p]  "w"
  [gen1p] -> Mux/1
  [gen2p] -> Mux/2
  [gen3p] -> Mux/3
  Bus Selector/1 -> [gen2w]  "<w>"
  Bus Selector1/1 -> [gen3w]  "<w>"
  Gen3@Bus3 PV 1.025 pu 85 MW/1(mGen) -> Bus Selector1/1, [mGen3]
  Gen1@Bus1 Swing/1(mGen) -> Bus Selector2/1, [mGen1]
  Bus Selector2/1 -> [gen1w]  "<w>"
  [gen1w] -> Mux/4
  [gen2w] -> Mux/5
  [gen3w] -> Mux/6
  Mux/1 -> To Workspace2/1
  PS-Simulink Converter6/1 -> [tielinep1]  "w"
  PS-Simulink Converter7/1 -> [tielinep2]  "w"
  [tielinep1] -> Mux3/1
  [tielinep2] -> Mux3/2
  Mux3/1 -> To Workspace3/1
  PS-Simulink Converter8/1 -> [loadp1]
  PS-Simulink Converter9/1 -> [loadp2]
  PS-Simulink Converter10/1 -> [loadp3]  "w"
  [loadp1] -> Mux1/1
  [loadp2] -> Mux1/2
  Mux1/1 -> To Workspace4/1
  [loadp3] -> Mux1/3
  PS-Simulink Converter3/1 -> [gen2p]
  [loadp1] -> To Workspace5/1
  PS-Simulink Converter11/1 -> [freqbus6]  "w"
  Frequency (Phasor)1/1 -> Scope3/1
  [freqbus6] -> Frequency (Phasor)2/1
  Frequency (Phasor)2/1 -> Scope4/1
  loadbus6p/1 -> Simulink-PS Converter4/1
  loadbus6q/1 -> Simulink-PS Converter5/1
  loadbus5q1/1 -> Simulink-PS Converter7/1
  loadbus5p1/1 -> Simulink-PS Converter6/1
  Step89/1 -> Simulink-PS Converter9/1
  Step46/1 -> Simulink-PS Converter8/1
  connections:
  Electrical Reference16/LConn1 -- Solver Configuration/RConn1 -- Load A 125 MW 50 MVAr/RConn1
  B7 to B8 50 km/RConn1 -- Bus8 230kV/LConn1
  B4 to B5 50 km/RConn1 -- Bus5 230kV/LConn2
  TF 7-2/LConn1 -- Bus7 230kV/LConn1
  B6 to B9 100 km/LConn2 -- Electrical Reference12/LConn1
  TF 4-1/LConn1 -- Bus4 230kV/LConn1
  Electrical Reference5/LConn1 -- B8 to B9 100 km/LConn2
  B7 to B8 50 km/RConn2 -- Electrical Reference4/LConn1
  TF 7-2/LConn2 -- Electrical Reference2/LConn1
  TF 9-3/LConn1 -- Bus9 230kV/LConn2
  TF 4-1/LConn2 -- Electrical Reference/LConn1
  B5 to B7 100 km/RConn2 -- Electrical Reference7/LConn1
  B5 to B7 100 km/LConn2 -- Electrical Reference8/LConn1
  B8 to B9 100 km/RConn2 -- Electrical Reference6/LConn1
  TF 9-3/LConn2 -- Electrical Reference1/LConn1
  B4 to B5 50 km/RConn2 -- Electrical Reference9/LConn1
  Electrical Reference3/LConn1 -- B7 to B8 50 km/LConn2
  B4 to B5 50 km/LConn2 -- Electrical Reference10/LConn1
  Electrical Reference17/LConn1 -- Load B 90 MW 30 MVAr/RConn1
  Electrical Reference15/LConn1 -- Load C 100 MW 35 MVAr/RConn1
  TF 4-1/RConn1 -- Bus1 16.5kV/RConn1
  Electrical Reference14/LConn1 -- B4 to B6 50 km/LConn2
  Electrical Reference13/LConn1 -- B4 to B6 50 km/RConn2
  Bus2 18kV/RConn1 -- TF 7-2/RConn1
  Bus6 230kV/LConn1 -- B6 to B9 100 km/LConn1
  B6 to B9 100 km/RConn2 -- Electrical Reference11/LConn1
  Circuit Breaker (Three-Phase)/LConn1 -- Simulink-PS Converter1/RConn1
  Electrical Reference18/LConn1 -- 50 MW/RConn1
  Circuit Breaker (Three-Phase)/RConn1 -- 50 MW/LConn1
  Bus6 230kV/RConn1 -- Circuit Breaker (Three-Phase)/LConn2
  Bus3 13.8kV/RConn1 -- TF 9-3/RConn1
  Bus7 230kV/RConn3 -- PS-Simulink Converter1/LConn1
  Simulink-PS Converter2/RConn1 -- Dynamic Load (Three-Phase)/LConn2
  Simulink-PS Converter3/RConn1 -- Dynamic Load (Three-Phase)/LConn3
  Bus7 230kV/RConn1 -- B5 to B7 100 km/RConn1
  PS-Simulink Converter6/LConn1 -- Power Sensor (Three-Phase)/LConn2
  B8 to B9 100 km/RConn1 -- Power Sensor (Three-Phase)/LConn1
  Power Sensor (Three-Phase)/RConn1 -- Bus9 230kV/LConn1
  PS-Simulink Converter7/LConn1 -- Power Sensor (Three-Phase)1/LConn2
  Power Sensor (Three-Phase)1/LConn1 -- B4 to B6 50 km/RConn1
  Power Sensor (Three-Phase)1/RConn1 -- Bus6 230kV/LConn2
  PS-Simulink Converter9/LConn1 -- Power Sensor (Three-Phase)2/LConn2
  Power Sensor (Three-Phase)2/LConn1 -- Bus6 230kV/RConn2
  Power Sensor (Three-Phase)3/LConn2 -- PS-Simulink Converter10/LConn1
  Power Sensor (Three-Phase)4/LConn1 -- Gen2@Bus2 PV 1.025 pu 163 MW/RConn1
  Power Sensor (Three-Phase)4/RConn1 -- Bus2 18kV/LConn1
  PS-Simulink Converter3/LConn1 -- Power Sensor (Three-Phase)4/LConn2
  Gen3@Bus3 PV 1.025 pu 85 MW/RConn1 -- Power Sensor (Three-Phase)5/LConn1
  Bus3 13.8kV/LConn1 -- Power Sensor (Three-Phase)5/RConn1
  PS-Simulink Converter4/LConn1 -- Power Sensor (Three-Phase)5/LConn2
  Power Sensor (Three-Phase)6/LConn1 -- Gen1@Bus1 Swing/RConn1
  Power Sensor (Three-Phase)6/RConn1 -- Bus1 16.5kV/LConn1
  PS-Simulink Converter5/LConn1 -- Power Sensor (Three-Phase)6/LConn2
  Bus8 230kV/RConn1 -- Power Sensor (Three-Phase)7/LConn1
  Power Sensor (Three-Phase)7/RConn1 -- Dynamic Load (Three-Phase)/LConn1
  PS-Simulink Converter8/LConn1 -- Power Sensor (Three-Phase)7/LConn2
  PS-Simulink Converter11/LConn1 -- Bus6 230kV/RConn4
  Load C 100 MW 35 MVAr/LConn1 -- Bus8 230kV/RConn2
  PS-Simulink Converter2/LConn1 -- Bus8 230kV/RConn4
  Simulink-PS Converter4/RConn1 -- Dynamic Load (Three-Phase)1/LConn2
  Simulink-PS Converter5/RConn1 -- Dynamic Load (Three-Phase)1/LConn3
  Dynamic Load (Three-Phase)1/LConn1 -- Power Sensor (Three-Phase)2/RConn1
  Simulink-PS Converter7/RConn1 -- Dynamic Load (Three-Phase)2/LConn3
  Simulink-PS Converter6/RConn1 -- Dynamic Load (Three-Phase)2/LConn2
  Circuit Breaker (Three-Phase)1/LConn2 -- Bus4 230kV/RConn1
  Circuit Breaker (Three-Phase)1/RConn1 -- B4 to B6 50 km/LConn1
  Simulink-PS Converter8/RConn1 -- Circuit Breaker (Three-Phase)1/LConn1
  Bus4 230kV/LConn2 -- B4 to B5 50 km/LConn1
  B5 to B7 100 km/LConn1 -- Bus5 230kV/LConn1
  B7 to B8 50 km/LConn1 -- Bus7 230kV/LConn2
  Circuit Breaker (Three-Phase)2/RConn1 -- B8 to B9 100 km/LConn1
  Circuit Breaker (Three-Phase)2/LConn2 -- Bus8 230kV/LConn2
  Simulink-PS Converter9/RConn1 -- Circuit Breaker (Three-Phase)2/LConn1
  Bus9 230kV/RConn1 -- B6 to B9 100 km/RConn1
  Power Sensor (Three-Phase)3/LConn1 -- Bus5 230kV/RConn1
  Power Sensor (Three-Phase)3/RConn1 -- Load A 125 MW 50 MVAr/LConn1
  Dynamic Load (Three-Phase)2/LConn1 -- Bus5 230kV/RConn2

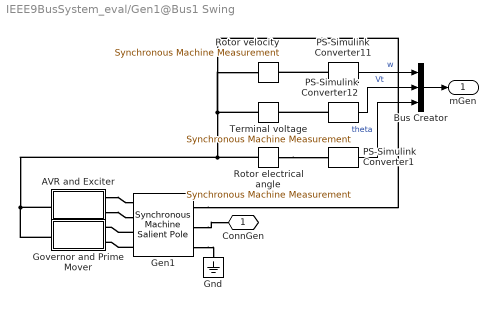
== system IEEE9BusSystem_eval/Gen1@Bus1 Swing ==
  AVR and Exciter : Subsystem
  Bus Creator : BusCreator  Inputs=3
  Gen1 : ee_lib/Electromechanical/Synchronous/Synchronous Machine Salient Pole  port_option=ee.enum.threePhasePort.composite  SRated=247.5 MW  VRated=16.5 kV  FRated=60 Hz  nPolePairs=20  param_option=ee.enum.sm.parameterization.standard  fieldCircuitParameterization_option=ee.enum.sm.fieldparameterization.current  baseEfd=100 V  baseIfd=100 A  zero_sequence=ee.enum.park.zerosequence.include  axes_param=ee.enum.rotorangle.qaxis  Ladu=0.2725  Laqu=0.1510  L0=0.0888  Ll=0.0888  Ra=0.01  Lfd=0.0817  Rfd=1.0656e-4  L1d=0.0121  R1d=0.0039  L1q=0.0265  R1q=0.0052  Xl=0.0832  Xd=0.3614  Xq=0.2398  X0=0.0832  Xdd=0.1505  Xddd=0.0990  Xqdd=0.1114  d_option=ee.enum.circuit.open  Td0d=8.96 s  Tdd=1.75 s  Td0dd=0.05 s  Tddd=0.0214 s  q_option=ee.enum.circuit.open  Tq0dd=0.09 s  Tqdd=0.0232 s  saturation_option=ee.enum.saturation.exclude  saturation_ifd=[0.0, 0.48, 0.76, 1.38, 1.79]  saturation_Vag=[0.0, 0.43, 0.59, 0.71, 0.76]  initialization_option=ee.enum.sm.initialization.steadystate  source_type=ee.enum.sm.load_flow_source_type.Swing  Vmag0=16.5*1.04 kV  Vang0=0 deg  Pt0=100e6 V*A  Qt0=0 V*A  minimum_pu=0.95  phase_search_range=[-30, 30] deg  gmin=1e-6 S  connection_option=ee.enum.Connection.wye  num_q_dampers=1  rotor_offset=-pi / 2 rad  pu_psid_specify=on  pu_psid_priority=High  pu_psid=0  pu_psid_nominal_specify=off  pu_psid_nominal_value=1  pu_psid_nominal_unit=1  pu_psiq_specify=on  pu_psiq_priority=High  pu_psiq=0  pu_psiq_nominal_specify=off  pu_psiq_nominal_value=1  pu_psiq_nominal_unit=1  pu_psifd_specify=on  pu_psifd_priority=High  pu_psifd=0  pu_psifd_nominal_specify=off  pu_psifd_nominal_value=1  pu_psifd_nominal_unit=1  pu_psi1d_specify=on  pu_psi1d_priority=High  pu_psi1d=0  pu_psi1d_nominal_specify=off  pu_psi1d_nominal_value=1  pu_psi1d_nominal_unit=1  pu_psi1q_specify=on  pu_psi1q_priority=High  pu_psi1q=0  pu_psi1q_nominal_specify=off  pu_psi1q_nominal_value=1  pu_psi1q_nominal_unit=1  angular_position_diff_specify=on  angular_position_diff_priority=High  angular_position_diff=-86.2419 deg  angular_position_diff_nominal_specify=off  angular_position_diff_nominal_value=1  angular_position_diff_nominal_unit=deg  Tmeas=298.15 K  alpha=3.93e-3 1/K  stator_thermal_mass=100 J/K  rotor_thermal_mass=200 J/K  temperatureA_specify=off  temperatureA_priority=High  temperatureA=25 degC  temperatureA_nominal_specify=off  temperatureA_nominal_value=1  temperatureA_nominal_unit=degC  temperatureB_specify=off  temperatureB_priority=High  temperatureB=25 degC  temperatureB_nominal_specify=off  temperatureB_nominal_value=1  temperatureB_nominal_unit=degC  temperatureC_specify=off  temperatureC_priority=High  temperatureC=25 degC  temperatureC_nominal_specify=off  temperatureC_nominal_value=1  temperatureC_nominal_unit=degC  temperatureR_specify=off  temperatureR_priority=High  temperatureR=25 degC  temperatureR_nominal_specify=off  temperatureR_nominal_value=1  temperatureR_nominal_unit=degC
      settings: InternalSimscapePortConfiguration="{\"Bottom\":[],\"Left\":[{\"id\":\"fd_p\",\"label\":\"fd+\",\"type\":\"foundation.electrical.electrical\"},{\"id\":\"fd_n\",\"label\":\"fd-\",\"type\":\"foundation.electrical.electrical\"},{\"id\":\"R\",\"label\":\"R\",\"type\":\"foundation.mechanical.rotational.rotational\"},{\"id\":\"C\",\"label\":\"C\",\"type\":\"foundation.mechanical.rotational.rotational\"}],\"Right\":[{\"id\":\"pu_output\",\"label\":\"pu\",\"type\":\"output\"},{\"id\":\"N\",\"label\":\"~\",\"type\":\"foundation.electrical.three_phase\"},{\"id\":\"n\",\"label\":\"n\",\"type\":\"foundation.electrical.electrical\"}],\"Top\":[]}"
  Gnd : fl_lib/Electrical/Electrical Elements/Electrical Reference
  Governor and Prime Mover : Subsystem
  PS-Simulink Converter1 : nesl_utility/PS-Simulink Converter  PhysicalDomain=network_engine_domain  SubClassName=ps_output  LeftPortType=input  RightPortType=output  PseudoPeriodic=off  Frequencies=[]  VectorFormat=1-D array  Unit=1  AffineConversion=off
  PS-Simulink Converter11 : nesl_utility/PS-Simulink Converter  PhysicalDomain=network_engine_domain  SubClassName=ps_output  LeftPortType=input  RightPortType=output  PseudoPeriodic=off  Frequencies=[]  VectorFormat=1-D array  Unit=1  AffineConversion=off
  PS-Simulink Converter12 : nesl_utility/PS-Simulink Converter  PhysicalDomain=network_engine_domain  SubClassName=ps_output  LeftPortType=input  RightPortType=output  PseudoPeriodic=off  Frequencies=[]  VectorFormat=1-D array  Unit=1  AffineConversion=off
  Rotor electrical angle : ee_lib/Electromechanical/Synchronous/Synchronous Machine Measurement  output_idx=19
      settings: InternalSimscapePortConfiguration="{\"Bottom\":[],\"Left\":[{\"id\":\"pu_input\",\"label\":\"pu\",\"type\":\"input\"}],\"Right\":[{\"id\":\"pu_output\",\"label\":\"o\",\"type\":\"output\"}],\"Top\":[]}"
  Rotor velocity : ee_lib/Electromechanical/Synchronous/Synchronous Machine Measurement  output_idx=4
      settings: InternalSimscapePortConfiguration="{\"Bottom\":[],\"Left\":[{\"id\":\"pu_input\",\"label\":\"pu\",\"type\":\"input\"}],\"Right\":[{\"id\":\"pu_output\",\"label\":\"o\",\"type\":\"output\"}],\"Top\":[]}"
  Terminal voltage : ee_lib/Electromechanical/Synchronous/Synchronous Machine Measurement  output_idx=14
      settings: InternalSimscapePortConfiguration="{\"Bottom\":[],\"Left\":[{\"id\":\"pu_input\",\"label\":\"pu\",\"type\":\"input\"}],\"Right\":[{\"id\":\"pu_output\",\"label\":\"o\",\"type\":\"output\"}],\"Top\":[]}"
  ConnGen : PMIOPort  Side=Right
  mGen : Outport
  wires:
  PS-Simulink Converter1/1 -> Bus Creator/3  "theta"
  PS-Simulink Converter12/1 -> Bus Creator/2  "Vt"
  Bus Creator/1 -> mGen/1
  PS-Simulink Converter11/1 -> Bus Creator/1  "w"
  connections:
  Rotor electrical angle/RConn1 -- PS-Simulink Converter1/LConn1
  PS-Simulink Converter12/LConn1 -- Terminal voltage/RConn1
  PS-Simulink Converter11/LConn1 -- Rotor velocity/RConn1
  Rotor electrical angle/LConn1 -- Gen1/RConn1 -- Rotor velocity/LConn1 -- Terminal voltage/LConn1 -- AVR and Exciter/LConn1 -- Governor and Prime Mover/LConn1
  Gen1/RConn3 -- Gnd/LConn1
  Gen1/RConn2 -- ConnGen/RConn1
  Gen1/LConn4 -- Governor and Prime Mover/RConn2
  Gen1/LConn3 -- Governor and Prime Mover/RConn1
  AVR and Exciter/RConn2 -- Gen1/LConn2
  AVR and Exciter/RConn1 -- Gen1/LConn1
